simulink model "s_c_nbe_m32k"  (R2018a)
settings: Solver=VariableStepDiscrete  StartTime=0.0  StopTime=1000  RelTol=1e-3
undefined symbols (not defined in the file): fft_stages, n_taps, output_bits, pfb_coeff_gen_calc, xengbits
libraries: xbsIndex_r4 x23714, casper_library_misc x17, xps_library x4, casper_library_scopes x4, xbsReplacements_r4 x4
(part 153 of 171)

== system s_c_nbe_m32k/nb_pfb/pfb_fir_generic1/pfb_fir_taps/tap_delays/rep_web0 ==
  in : Inport
  bussify : Subsystem  mask(bus_create){inputNum=108}
      mask prompts: inputNum "Number of inputs:"
      mask init:
      | bus_create_init(gcb,...
      |     'inputNum', inputNum);
  din0_0 : xbsIndex_r4/Delay  rst=off  infoeditControl=Selection of Reset will increase slice count due to use of real FFs and instead of SRLs  en=off  latency=1  reg_retiming=off  dbl_ovrd=off  block_type=delay
  din0_1 : xbsIndex_r4/Delay  rst=off  infoeditControl=Selection of Reset will increase slice count due to use of real FFs and instead of SRLs  en=off  latency=1  reg_retiming=off  dbl_ovrd=off  block_type=delay
  din0_2 : xbsIndex_r4/Delay  rst=off  infoeditControl=Selection of Reset will increase slice count due to use of real FFs and instead of SRLs  en=off  latency=1  reg_retiming=off  dbl_ovrd=off  block_type=delay
  din1_{0..11} (12 alike) : xbsIndex_r4/Delay  rst=off  infoeditControl=Selection of Reset will increase slice count due to use of real FFs and instead of SRLs  en=off  latency=1  reg_retiming=off  dbl_ovrd=off  block_type=delay
  din2_{0..47} (48 alike) : xbsIndex_r4/Delay  rst=off  infoeditControl=Selection of Reset will increase slice count due to use of real FFs and instead of SRLs  en=off  latency=1  reg_retiming=off  dbl_ovrd=off  block_type=delay
  din3_{0..107} (108 alike) : xbsIndex_r4/Delay  rst=off  infoeditControl=Selection of Reset will increase slice count due to use of real FFs and instead of SRLs  en=off  latency=1  reg_retiming=off  dbl_ovrd=off  block_type=delay
  out : Outport
  wires:
  in/1 -> din0_0/1, din0_1/1, din0_2/1
  din0_0/1 -> din1_0/1, din1_3/1, din1_6/1, din1_9/1
  din0_1/1 -> din1_1/1, din1_4/1, din1_7/1, din1_10/1
  din0_2/1 -> din1_2/1, din1_5/1, din1_8/1, din1_11/1
  din1_0/1 -> din2_0/1, din2_12/1, din2_24/1, din2_36/1
  din1_1/1 -> din2_1/1, din2_13/1, din2_25/1, din2_37/1
  din1_2/1 -> din2_2/1, din2_14/1, din2_26/1, din2_38/1
  din1_3/1 -> din2_3/1, din2_15/1, din2_27/1, din2_39/1
  din1_4/1 -> din2_4/1, din2_16/1, din2_28/1, din2_40/1
  din1_5/1 -> din2_5/1, din2_17/1, din2_29/1, din2_41/1
  din1_6/1 -> din2_6/1, din2_18/1, din2_30/1, din2_42/1
  din1_7/1 -> din2_7/1, din2_19/1, din2_31/1, din2_43/1
  din1_8/1 -> din2_8/1, din2_20/1, din2_32/1, din2_44/1
  din1_9/1 -> din2_9/1, din2_21/1, din2_33/1, din2_45/1
  din1_10/1 -> din2_10/1, din2_22/1, din2_34/1, din2_46/1
  din1_11/1 -> din2_11/1, din2_23/1, din2_35/1, din2_47/1
  din2_0/1 -> din3_0/1, din3_48/1, din3_96/1
  din2_1/1 -> din3_1/1, din3_49/1, din3_97/1
  din2_2/1 -> din3_2/1, din3_50/1, din3_98/1
  din2_3/1 -> din3_3/1, din3_51/1, din3_99/1
  din2_4/1 -> din3_4/1, din3_52/1, din3_100/1
  din2_5/1 -> din3_5/1, din3_53/1, din3_101/1
  din2_6/1 -> din3_6/1, din3_54/1, din3_102/1
  din2_7/1 -> din3_7/1, din3_55/1, din3_103/1
  din2_8/1 -> din3_8/1, din3_56/1, din3_104/1
  din2_9/1 -> din3_9/1, din3_57/1, din3_105/1
  din2_10/1 -> din3_10/1, din3_58/1, din3_106/1
  din2_11/1 -> din3_11/1, din3_59/1, din3_107/1
  din2_12/1 -> din3_12/1, din3_60/1
  din2_13/1 -> din3_13/1, din3_61/1
  din2_14/1 -> din3_14/1, din3_62/1
  din2_15/1 -> din3_15/1, din3_63/1
  din2_16/1 -> din3_16/1, din3_64/1
  din2_17/1 -> din3_17/1, din3_65/1
  din2_18/1 -> din3_18/1, din3_66/1
  din2_19/1 -> din3_19/1, din3_67/1
  din2_20/1 -> din3_20/1, din3_68/1
  din2_21/1 -> din3_21/1, din3_69/1
  din2_22/1 -> din3_22/1, din3_70/1
  din2_23/1 -> din3_23/1, din3_71/1
  din2_24/1 -> din3_24/1, din3_72/1
  din2_25/1 -> din3_25/1, din3_73/1
  din2_26/1 -> din3_26/1, din3_74/1
  din2_27/1 -> din3_27/1, din3_75/1
  din2_28/1 -> din3_28/1, din3_76/1
  din2_29/1 -> din3_29/1, din3_77/1
  din2_30/1 -> din3_30/1, din3_78/1
  din2_31/1 -> din3_31/1, din3_79/1
  din2_32/1 -> din3_32/1, din3_80/1
  din2_33/1 -> din3_33/1, din3_81/1
  din2_34/1 -> din3_34/1, din3_82/1
  din2_35/1 -> din3_35/1, din3_83/1
  din2_36/1 -> din3_36/1, din3_84/1
  din2_37/1 -> din3_37/1, din3_85/1
  din2_38/1 -> din3_38/1, din3_86/1
  din2_39/1 -> din3_39/1, din3_87/1
  din2_40/1 -> din3_40/1, din3_88/1
  din2_41/1 -> din3_41/1, din3_89/1
  din2_42/1 -> din3_42/1, din3_90/1
  din2_43/1 -> din3_43/1, din3_91/1
  din2_44/1 -> din3_44/1, din3_92/1
  din2_45/1 -> din3_45/1, din3_93/1
  din2_46/1 -> din3_46/1, din3_94/1
  din2_47/1 -> din3_47/1, din3_95/1
  din3_0/1 -> bussify/1(in1)
  din3_1/1 -> bussify/2(in2)
  din3_2/1 -> bussify/3(in3)
  din3_3/1 -> bussify/4(in4)
  din3_4/1 -> bussify/5(in5)
  din3_5/1 -> bussify/6(in6)
  din3_6/1 -> bussify/7(in7)
  din3_7/1 -> bussify/8(in8)
  din3_8/1 -> bussify/9(in9)
  din3_9/1 -> bussify/10(in10)
  din3_10/1 -> bussify/11(in11)
  din3_11/1 -> bussify/12(in12)
  din3_12/1 -> bussify/13(in13)
  din3_13/1 -> bussify/14(in14)
  din3_14/1 -> bussify/15(in15)
  din3_15/1 -> bussify/16(in16)
  din3_16/1 -> bussify/17(in17)
  din3_17/1 -> bussify/18(in18)
  din3_18/1 -> bussify/19(in19)
  din3_19/1 -> bussify/20(in20)
  din3_20/1 -> bussify/21(in21)
  din3_21/1 -> bussify/22(in22)
  din3_22/1 -> bussify/23(in23)
  din3_23/1 -> bussify/24(in24)
  din3_24/1 -> bussify/25(in25)
  din3_25/1 -> bussify/26(in26)
  din3_26/1 -> bussify/27(in27)
  din3_27/1 -> bussify/28(in28)
  din3_28/1 -> bussify/29(in29)
  din3_29/1 -> bussify/30(in30)
  din3_30/1 -> bussify/31(in31)
  din3_31/1 -> bussify/32(in32)
  din3_32/1 -> bussify/33(in33)
  din3_33/1 -> bussify/34(in34)
  din3_34/1 -> bussify/35(in35)
  din3_35/1 -> bussify/36(in36)
  din3_36/1 -> bussify/37(in37)
  din3_37/1 -> bussify/38(in38)
  din3_38/1 -> bussify/39(in39)
  din3_39/1 -> bussify/40(in40)
  din3_40/1 -> bussify/41(in41)
  din3_41/1 -> bussify/42(in42)
  din3_42/1 -> bussify/43(in43)
  din3_43/1 -> bussify/44(in44)
  din3_44/1 -> bussify/45(in45)
  din3_45/1 -> bussify/46(in46)
  din3_46/1 -> bussify/47(in47)
  din3_47/1 -> bussify/48(in48)
  din3_48/1 -> bussify/49(in49)
  din3_49/1 -> bussify/50(in50)
  din3_50/1 -> bussify/51(in51)
  din3_51/1 -> bussify/52(in52)
  din3_52/1 -> bussify/53(in53)
  din3_53/1 -> bussify/54(in54)
  din3_54/1 -> bussify/55(in55)
  din3_55/1 -> bussify/56(in56)
  din3_56/1 -> bussify/57(in57)
  din3_57/1 -> bussify/58(in58)
  din3_58/1 -> bussify/59(in59)
  din3_59/1 -> bussify/60(in60)
  din3_60/1 -> bussify/61(in61)
  din3_61/1 -> bussify/62(in62)
  din3_62/1 -> bussify/63(in63)
  din3_63/1 -> bussify/64(in64)
  din3_64/1 -> bussify/65(in65)
  din3_65/1 -> bussify/66(in66)
  din3_66/1 -> bussify/67(in67)
  din3_67/1 -> bussify/68(in68)
  din3_68/1 -> bussify/69(in69)
  din3_69/1 -> bussify/70(in70)
  din3_70/1 -> bussify/71(in71)
  din3_71/1 -> bussify/72(in72)
  din3_72/1 -> bussify/73(in73)
  din3_73/1 -> bussify/74(in74)
  din3_74/1 -> bussify/75(in75)
  din3_75/1 -> bussify/76(in76)
  din3_76/1 -> bussify/77(in77)
  din3_77/1 -> bussify/78(in78)
  din3_78/1 -> bussify/79(in79)
  din3_79/1 -> bussify/80(in80)
  din3_80/1 -> bussify/81(in81)
  din3_81/1 -> bussify/82(in82)
  din3_82/1 -> bussify/83(in83)
  din3_83/1 -> bussify/84(in84)
  din3_84/1 -> bussify/85(in85)
  din3_85/1 -> bussify/86(in86)
  din3_86/1 -> bussify/87(in87)
  din3_87/1 -> bussify/88(in88)
  din3_88/1 -> bussify/89(in89)
  din3_89/1 -> bussify/90(in90)
  din3_90/1 -> bussify/91(in91)
  din3_91/1 -> bussify/92(in92)
  din3_92/1 -> bussify/93(in93)
  din3_93/1 -> bussify/94(in94)
  din3_94/1 -> bussify/95(in95)
  din3_95/1 -> bussify/96(in96)
  din3_96/1 -> bussify/97(in97)
  din3_97/1 -> bussify/98(in98)
  din3_98/1 -> bussify/99(in99)
  din3_99/1 -> bussify/100(in100)
  din3_100/1 -> bussify/101(in101)
  din3_101/1 -> bussify/102(in102)
  din3_102/1 -> bussify/103(in103)
  din3_103/1 -> bussify/104(in104)
  din3_104/1 -> bussify/105(in105)
  din3_105/1 -> bussify/106(in106)
  din3_106/1 -> bussify/107(in107)
  din3_107/1 -> bussify/108(in108)
  bussify/1(bus_out) -> out/1

== system s_c_nbe_m32k/nb_pfb/pfb_fir_generic2/pfb_fir_coeff_gen/munge/join ==
  in1 : Inport
  in2 : Inport  Port=2
  concatenate : xbsIndex_r4/Concat  num_inputs=2  dbl_ovrd=off  block_type=concat
  reinterpret1 : xbsIndex_r4/Reinterpret  force_arith_type=on  arith_type=Unsigned  force_bin_pt=on  bin_pt=0  block_type=reinterpret
      settings: infoedit="Changes signal type without altering the binary representation.   You can changed the signal between signed and unsigned, and relocate the binary point.<br><br>Hardware notes: In hardware this block costs nothing.<br><br>Example:  Suppose the input is 6 bits wide, signed, with 2 fractional bits, and the output is forced to unsigned with 0 fractional bits.  Then an input of -2.0 (1110.00 in binary 2's complement) becomes an output of 56 (111000 in binary)."
  reinterpret2 : xbsIndex_r4/Reinterpret  force_arith_type=on  arith_type=Unsigned  force_bin_pt=on  bin_pt=0  block_type=reinterpret
      settings: infoedit="Changes signal type without altering the binary representation.   You can changed the signal between signed and unsigned, and relocate the binary point.<br><br>Hardware notes: In hardware this block costs nothing.<br><br>Example:  Suppose the input is 6 bits wide, signed, with 2 fractional bits, and the output is forced to unsigned with 0 fractional bits.  Then an input of -2.0 (1110.00 in binary 2's complement) becomes an output of 56 (111000 in binary)."
  bus_out : Outport
  wires:
  concatenate/1 -> bus_out/1
  in1/1 -> reinterpret1/1
  reinterpret1/1 -> concatenate/1
  in2/1 -> reinterpret2/1
  reinterpret2/1 -> concatenate/2

== system s_c_nbe_m32k/nb_pfb/pfb_fir_generic2/pfb_fir_coeff_gen/munge/split ==
  bus_in : Inport
  reinterpret1 : xbsIndex_r4/Reinterpret  force_arith_type=on  arith_type=Unsigned  force_bin_pt=on  bin_pt=0  block_type=reinterpret
  reinterpret2 : xbsIndex_r4/Reinterpret  force_arith_type=on  arith_type=Unsigned  force_bin_pt=on  bin_pt=0  block_type=reinterpret
  slice1 : xbsIndex_r4/Slice  nbits=18  boolean_output=off  mode=Upper Bit Location + Width  bit1=-18  base1=MSB of Input  bit0=0  base0=LSB of Input  dbl_ovrd=off  block_type=slice
  slice2 : xbsIndex_r4/Slice  nbits=18  boolean_output=off  mode=Upper Bit Location + Width  bit1=0  base1=MSB of Input  bit0=0  base0=LSB of Input  dbl_ovrd=off  block_type=slice
  msb_out2 : Outport
  lsb_out1 : Outport  Port=2
  wires:
  bus_in/1 -> slice2/1, slice1/1
  slice2/1 -> reinterpret2/1
  reinterpret2/1 -> msb_out2/1
  slice1/1 -> reinterpret1/1
  reinterpret1/1 -> lsb_out1/1

== system s_c_nbe_m32k/nb_pfb/pfb_fir_generic2/pfb_fir_coeff_gen/rom/A_bussify0 ==
  in1 : Inport
  in2 : Inport  Port=2
  in3 : Inport  Port=3
  in4 : Inport  Port=4
  in5 : Inport  Port=5
  in6 : Inport  Port=6
  in7 : Inport  Port=7
  in8 : Inport  Port=8
  in9 : Inport  Port=9
  in10 : Inport  Port=10
  in11 : Inport  Port=11
  in12 : Inport  Port=12
  in13 : Inport  Port=13
  in14 : Inport  Port=14
  in15 : Inport  Port=15
  in16 : Inport  Port=16
  in17 : Inport  Port=17
  in18 : Inport  Port=18
  in19 : Inport  Port=19
  in20 : Inport  Port=20
  in21 : Inport  Port=21
  in22 : Inport  Port=22
  in23 : Inport  Port=23
  in24 : Inport  Port=24
  in25 : Inport  Port=25
  in26 : Inport  Port=26
  in27 : Inport  Port=27
  in28 : Inport  Port=28
  in29 : Inport  Port=29
  in30 : Inport  Port=30
  in31 : Inport  Port=31
  in32 : Inport  Port=32
  in33 : Inport  Port=33
  in34 : Inport  Port=34
  in35 : Inport  Port=35
  in36 : Inport  Port=36
  concatenate : xbsIndex_r4/Concat  num_inputs=36  dbl_ovrd=off  block_type=concat
  reinterpret{1..36} (36 alike) : xbsIndex_r4/Reinterpret  force_arith_type=on  arith_type=Unsigned  force_bin_pt=on  bin_pt=0  block_type=reinterpret
      reinterpret1 settings: infoedit="Changes signal type without altering the binary representation.   You can changed the signal between signed and unsigned, and relocate the binary point.<br><br>Hardware notes: In hardware this block costs nothing.<br><br>Example:  Suppose the input is 6 bits wide, signed, with 2 fractional bits, and the output is forced to unsigned with 0 fractional bits.  Then an input of -2.0 (1110.00 in binary 2's complement) becomes an output of 56 (111000 in binary)."
      reinterpret2 settings: infoedit="Changes signal type without altering the binary representation.   You can changed the signal between signed and unsigned, and relocate the binary point.<br><br>Hardware notes: In hardware this block costs nothing.<br><br>Example:  Suppose the input is 6 bits wide, signed, with 2 fractional bits, and the output is forced to unsigned with 0 fractional bits.  Then an input of -2.0 (1110.00 in binary 2's complement) becomes an output of 56 (111000 in binary)."
  bus_out : Outport
  wires:
  concatenate/1 -> bus_out/1
  in1/1 -> reinterpret1/1
  reinterpret1/1 -> concatenate/1
  in2/1 -> reinterpret2/1
  reinterpret2/1 -> concatenate/2
  in3/1 -> reinterpret3/1
  reinterpret3/1 -> concatenate/3
  in4/1 -> reinterpret4/1
  reinterpret4/1 -> concatenate/4
  in5/1 -> reinterpret5/1
  reinterpret5/1 -> concatenate/5
  in6/1 -> reinterpret6/1
  reinterpret6/1 -> concatenate/6
  in7/1 -> reinterpret7/1
  reinterpret7/1 -> concatenate/7
  in8/1 -> reinterpret8/1
  reinterpret8/1 -> concatenate/8
  in9/1 -> reinterpret9/1
  reinterpret9/1 -> concatenate/9
  in10/1 -> reinterpret10/1
  reinterpret10/1 -> concatenate/10
  in11/1 -> reinterpret11/1
  reinterpret11/1 -> concatenate/11
  in12/1 -> reinterpret12/1
  reinterpret12/1 -> concatenate/12
  in13/1 -> reinterpret13/1
  reinterpret13/1 -> concatenate/13
  in14/1 -> reinterpret14/1
  reinterpret14/1 -> concatenate/14
  in15/1 -> reinterpret15/1
  reinterpret15/1 -> concatenate/15
  in16/1 -> reinterpret16/1
  reinterpret16/1 -> concatenate/16
  in17/1 -> reinterpret17/1
  reinterpret17/1 -> concatenate/17
  in18/1 -> reinterpret18/1
  reinterpret18/1 -> concatenate/18
  in19/1 -> reinterpret19/1
  reinterpret19/1 -> concatenate/19
  in20/1 -> reinterpret20/1
  reinterpret20/1 -> concatenate/20
  in21/1 -> reinterpret21/1
  reinterpret21/1 -> concatenate/21
  in22/1 -> reinterpret22/1
  reinterpret22/1 -> concatenate/22
  in23/1 -> reinterpret23/1
  reinterpret23/1 -> concatenate/23
  in24/1 -> reinterpret24/1
  reinterpret24/1 -> concatenate/24
  in25/1 -> reinterpret25/1
  reinterpret25/1 -> concatenate/25
  in26/1 -> reinterpret26/1
  reinterpret26/1 -> concatenate/26
  in27/1 -> reinterpret27/1
  reinterpret27/1 -> concatenate/27
  in28/1 -> reinterpret28/1
  reinterpret28/1 -> concatenate/28
  in29/1 -> reinterpret29/1
  reinterpret29/1 -> concatenate/29
  in30/1 -> reinterpret30/1
  reinterpret30/1 -> concatenate/30
  in31/1 -> reinterpret31/1
  reinterpret31/1 -> concatenate/31
  in32/1 -> reinterpret32/1
  reinterpret32/1 -> concatenate/32
  in33/1 -> reinterpret33/1
  reinterpret33/1 -> concatenate/33
  in34/1 -> reinterpret34/1
  reinterpret34/1 -> concatenate/34
  in35/1 -> reinterpret35/1
  reinterpret35/1 -> concatenate/35
  in36/1 -> reinterpret36/1
  reinterpret36/1 -> concatenate/36

== system s_c_nbe_m32k/nb_pfb/pfb_fir_generic2/pfb_fir_coeff_gen/rom/B_bussify0 ==
  in1 : Inport
  in2 : Inport  Port=2
  in3 : Inport  Port=3
  in4 : Inport  Port=4
  in5 : Inport  Port=5
  in6 : Inport  Port=6
  in7 : Inport  Port=7
  in8 : Inport  Port=8
  in9 : Inport  Port=9
  in10 : Inport  Port=10
  in11 : Inport  Port=11
  in12 : Inport  Port=12
  in13 : Inport  Port=13
  in14 : Inport  Port=14
  in15 : Inport  Port=15
  in16 : Inport  Port=16
  in17 : Inport  Port=17
  in18 : Inport  Port=18
  in19 : Inport  Port=19
  in20 : Inport  Port=20
  in21 : Inport  Port=21
  in22 : Inport  Port=22
  in23 : Inport  Port=23
  in24 : Inport  Port=24
  in25 : Inport  Port=25
  in26 : Inport  Port=26
  in27 : Inport  Port=27
  in28 : Inport  Port=28
  in29 : Inport  Port=29
  in30 : Inport  Port=30
  in31 : Inport  Port=31
  in32 : Inport  Port=32
  in33 : Inport  Port=33
  in34 : Inport  Port=34
  in35 : Inport  Port=35
  in36 : Inport  Port=36
  concatenate : xbsIndex_r4/Concat  num_inputs=36  dbl_ovrd=off  block_type=concat
  reinterpret{1..36} (36 alike) : xbsIndex_r4/Reinterpret  force_arith_type=on  arith_type=Unsigned  force_bin_pt=on  bin_pt=0  block_type=reinterpret
      reinterpret1 settings: infoedit="Changes signal type without altering the binary representation.   You can changed the signal between signed and unsigned, and relocate the binary point.<br><br>Hardware notes: In hardware this block costs nothing.<br><br>Example:  Suppose the input is 6 bits wide, signed, with 2 fractional bits, and the output is forced to unsigned with 0 fractional bits.  Then an input of -2.0 (1110.00 in binary 2's complement) becomes an output of 56 (111000 in binary)."
      reinterpret2 settings: infoedit="Changes signal type without altering the binary representation.   You can changed the signal between signed and unsigned, and relocate the binary point.<br><br>Hardware notes: In hardware this block costs nothing.<br><br>Example:  Suppose the input is 6 bits wide, signed, with 2 fractional bits, and the output is forced to unsigned with 0 fractional bits.  Then an input of -2.0 (1110.00 in binary 2's complement) becomes an output of 56 (111000 in binary)."
  bus_out : Outport
  wires:
  concatenate/1 -> bus_out/1
  in1/1 -> reinterpret1/1
  reinterpret1/1 -> concatenate/1
  in2/1 -> reinterpret2/1
  reinterpret2/1 -> concatenate/2
  in3/1 -> reinterpret3/1
  reinterpret3/1 -> concatenate/3
  in4/1 -> reinterpret4/1
  reinterpret4/1 -> concatenate/4
  in5/1 -> reinterpret5/1
  reinterpret5/1 -> concatenate/5
  in6/1 -> reinterpret6/1
  reinterpret6/1 -> concatenate/6
  in7/1 -> reinterpret7/1
  reinterpret7/1 -> concatenate/7
  in8/1 -> reinterpret8/1
  reinterpret8/1 -> concatenate/8
  in9/1 -> reinterpret9/1
  reinterpret9/1 -> concatenate/9
  in10/1 -> reinterpret10/1
  reinterpret10/1 -> concatenate/10
  in11/1 -> reinterpret11/1
  reinterpret11/1 -> concatenate/11
  in12/1 -> reinterpret12/1
  reinterpret12/1 -> concatenate/12
  in13/1 -> reinterpret13/1
  reinterpret13/1 -> concatenate/13
  in14/1 -> reinterpret14/1
  reinterpret14/1 -> concatenate/14
  in15/1 -> reinterpret15/1
  reinterpret15/1 -> concatenate/15
  in16/1 -> reinterpret16/1
  reinterpret16/1 -> concatenate/16
  in17/1 -> reinterpret17/1
  reinterpret17/1 -> concatenate/17
  in18/1 -> reinterpret18/1
  reinterpret18/1 -> concatenate/18
  in19/1 -> reinterpret19/1
  reinterpret19/1 -> concatenate/19
  in20/1 -> reinterpret20/1
  reinterpret20/1 -> concatenate/20
  in21/1 -> reinterpret21/1
  reinterpret21/1 -> concatenate/21
  in22/1 -> reinterpret22/1
  reinterpret22/1 -> concatenate/22
  in23/1 -> reinterpret23/1
  reinterpret23/1 -> concatenate/23
  in24/1 -> reinterpret24/1
  reinterpret24/1 -> concatenate/24
  in25/1 -> reinterpret25/1
  reinterpret25/1 -> concatenate/25
  in26/1 -> reinterpret26/1
  reinterpret26/1 -> concatenate/26
  in27/1 -> reinterpret27/1
  reinterpret27/1 -> concatenate/27
  in28/1 -> reinterpret28/1
  reinterpret28/1 -> concatenate/28
  in29/1 -> reinterpret29/1
  reinterpret29/1 -> concatenate/29
  in30/1 -> reinterpret30/1
  reinterpret30/1 -> concatenate/30
  in31/1 -> reinterpret31/1
  reinterpret31/1 -> concatenate/31
  in32/1 -> reinterpret32/1
  reinterpret32/1 -> concatenate/32
  in33/1 -> reinterpret33/1
  reinterpret33/1 -> concatenate/33
  in34/1 -> reinterpret34/1
  reinterpret34/1 -> concatenate/34
  in35/1 -> reinterpret35/1
  reinterpret35/1 -> concatenate/35
  in36/1 -> reinterpret36/1
  reinterpret36/1 -> concatenate/36

== system s_c_nbe_m32k/nb_pfb/pfb_fir_generic2/pfb_fir_coeff_gen/rom/debus_addra0 ==
  bus_in : Inport
  reinterpret{1..36} (36 alike) : xbsIndex_r4/Reinterpret  force_arith_type=on  arith_type=Unsigned  force_bin_pt=on  bin_pt=0  block_type=reinterpret
  slice1 : xbsIndex_r4/Slice  nbits=15  boolean_output=off  mode=Upper Bit Location + Width  bit1=-525  base1=MSB of Input  bit0=0  base0=LSB of Input  dbl_ovrd=off  block_type=slice
  slice10 : xbsIndex_r4/Slice  nbits=15  boolean_output=off  mode=Upper Bit Location + Width  bit1=-390  base1=MSB of Input  bit0=0  base0=LSB of Input  dbl_ovrd=off  block_type=slice
  slice11 : xbsIndex_r4/Slice  nbits=15  boolean_output=off  mode=Upper Bit Location + Width  bit1=-375  base1=MSB of Input  bit0=0  base0=LSB of Input  dbl_ovrd=off  block_type=slice
  slice12 : xbsIndex_r4/Slice  nbits=15  boolean_output=off  mode=Upper Bit Location + Width  bit1=-360  base1=MSB of Input  bit0=0  base0=LSB of Input  dbl_ovrd=off  block_type=slice
  slice13 : xbsIndex_r4/Slice  nbits=15  boolean_output=off  mode=Upper Bit Location + Width  bit1=-345  base1=MSB of Input  bit0=0  base0=LSB of Input  dbl_ovrd=off  block_type=slice
  slice14 : xbsIndex_r4/Slice  nbits=15  boolean_output=off  mode=Upper Bit Location + Width  bit1=-330  base1=MSB of Input  bit0=0  base0=LSB of Input  dbl_ovrd=off  block_type=slice
  slice15 : xbsIndex_r4/Slice  nbits=15  boolean_output=off  mode=Upper Bit Location + Width  bit1=-315  base1=MSB of Input  bit0=0  base0=LSB of Input  dbl_ovrd=off  block_type=slice
  slice16 : xbsIndex_r4/Slice  nbits=15  boolean_output=off  mode=Upper Bit Location + Width  bit1=-300  base1=MSB of Input  bit0=0  base0=LSB of Input  dbl_ovrd=off  block_type=slice
  slice17 : xbsIndex_r4/Slice  nbits=15  boolean_output=off  mode=Upper Bit Location + Width  bit1=-285  base1=MSB of Input  bit0=0  base0=LSB of Input  dbl_ovrd=off  block_type=slice
  slice18 : xbsIndex_r4/Slice  nbits=15  boolean_output=off  mode=Upper Bit Location + Width  bit1=-270  base1=MSB of Input  bit0=0  base0=LSB of Input  dbl_ovrd=off  block_type=slice
  slice19 : xbsIndex_r4/Slice  nbits=15  boolean_output=off  mode=Upper Bit Location + Width  bit1=-255  base1=MSB of Input  bit0=0  base0=LSB of Input  dbl_ovrd=off  block_type=slice
  slice2 : xbsIndex_r4/Slice  nbits=15  boolean_output=off  mode=Upper Bit Location + Width  bit1=-510  base1=MSB of Input  bit0=0  base0=LSB of Input  dbl_ovrd=off  block_type=slice
  slice20 : xbsIndex_r4/Slice  nbits=15  boolean_output=off  mode=Upper Bit Location + Width  bit1=-240  base1=MSB of Input  bit0=0  base0=LSB of Input  dbl_ovrd=off  block_type=slice
  slice21 : xbsIndex_r4/Slice  nbits=15  boolean_output=off  mode=Upper Bit Location + Width  bit1=-225  base1=MSB of Input  bit0=0  base0=LSB of Input  dbl_ovrd=off  block_type=slice
  slice22 : xbsIndex_r4/Slice  nbits=15  boolean_output=off  mode=Upper Bit Location + Width  bit1=-210  base1=MSB of Input  bit0=0  base0=LSB of Input  dbl_ovrd=off  block_type=slice
  slice23 : xbsIndex_r4/Slice  nbits=15  boolean_output=off  mode=Upper Bit Location + Width  bit1=-195  base1=MSB of Input  bit0=0  base0=LSB of Input  dbl_ovrd=off  block_type=slice
  slice24 : xbsIndex_r4/Slice  nbits=15  boolean_output=off  mode=Upper Bit Location + Width  bit1=-180  base1=MSB of Input  bit0=0  base0=LSB of Input  dbl_ovrd=off  block_type=slice
  slice25 : xbsIndex_r4/Slice  nbits=15  boolean_output=off  mode=Upper Bit Location + Width  bit1=-165  base1=MSB of Input  bit0=0  base0=LSB of Input  dbl_ovrd=off  block_type=slice
  slice26 : xbsIndex_r4/Slice  nbits=15  boolean_output=off  mode=Upper Bit Location + Width  bit1=-150  base1=MSB of Input  bit0=0  base0=LSB of Input  dbl_ovrd=off  block_type=slice
  slice27 : xbsIndex_r4/Slice  nbits=15  boolean_output=off  mode=Upper Bit Location + Width  bit1=-135  base1=MSB of Input  bit0=0  base0=LSB of Input  dbl_ovrd=off  block_type=slice
  slice28 : xbsIndex_r4/Slice  nbits=15  boolean_output=off  mode=Upper Bit Location + Width  bit1=-120  base1=MSB of Input  bit0=0  base0=LSB of Input  dbl_ovrd=off  block_type=slice
  slice29 : xbsIndex_r4/Slice  nbits=15  boolean_output=off  mode=Upper Bit Location + Width  bit1=-105  base1=MSB of Input  bit0=0  base0=LSB of Input  dbl_ovrd=off  block_type=slice
  slice3 : xbsIndex_r4/Slice  nbits=15  boolean_output=off  mode=Upper Bit Location + Width  bit1=-495  base1=MSB of Input  bit0=0  base0=LSB of Input  dbl_ovrd=off  block_type=slice
  slice30 : xbsIndex_r4/Slice  nbits=15  boolean_output=off  mode=Upper Bit Location + Width  bit1=-90  base1=MSB of Input  bit0=0  base0=LSB of Input  dbl_ovrd=off  block_type=slice
  slice31 : xbsIndex_r4/Slice  nbits=15  boolean_output=off  mode=Upper Bit Location + Width  bit1=-75  base1=MSB of Input  bit0=0  base0=LSB of Input  dbl_ovrd=off  block_type=slice
  slice32 : xbsIndex_r4/Slice  nbits=15  boolean_output=off  mode=Upper Bit Location + Width  bit1=-60  base1=MSB of Input  bit0=0  base0=LSB of Input  dbl_ovrd=off  block_type=slice
  slice33 : xbsIndex_r4/Slice  nbits=15  boolean_output=off  mode=Upper Bit Location + Width  bit1=-45  base1=MSB of Input  bit0=0  base0=LSB of Input  dbl_ovrd=off  block_type=slice
  slice34 : xbsIndex_r4/Slice  nbits=15  boolean_output=off  mode=Upper Bit Location + Width  bit1=-30  base1=MSB of Input  bit0=0  base0=LSB of Input  dbl_ovrd=off  block_type=slice
  slice35 : xbsIndex_r4/Slice  nbits=15  boolean_output=off  mode=Upper Bit Location + Width  bit1=-15  base1=MSB of Input  bit0=0  base0=LSB of Input  dbl_ovrd=off  block_type=slice
  slice36 : xbsIndex_r4/Slice  nbits=15  boolean_output=off  mode=Upper Bit Location + Width  bit1=0  base1=MSB of Input  bit0=0  base0=LSB of Input  dbl_ovrd=off  block_type=slice
  slice4 : xbsIndex_r4/Slice  nbits=15  boolean_output=off  mode=Upper Bit Location + Width  bit1=-480  base1=MSB of Input  bit0=0  base0=LSB of Input  dbl_ovrd=off  block_type=slice
  slice5 : xbsIndex_r4/Slice  nbits=15  boolean_output=off  mode=Upper Bit Location + Width  bit1=-465  base1=MSB of Input  bit0=0  base0=LSB of Input  dbl_ovrd=off  block_type=slice
  slice6 : xbsIndex_r4/Slice  nbits=15  boolean_output=off  mode=Upper Bit Location + Width  bit1=-450  base1=MSB of Input  bit0=0  base0=LSB of Input  dbl_ovrd=off  block_type=slice
  slice7 : xbsIndex_r4/Slice  nbits=15  boolean_output=off  mode=Upper Bit Location + Width  bit1=-435  base1=MSB of Input  bit0=0  base0=LSB of Input  dbl_ovrd=off  block_type=slice
  slice8 : xbsIndex_r4/Slice  nbits=15  boolean_output=off  mode=Upper Bit Location + Width  bit1=-420  base1=MSB of Input  bit0=0  base0=LSB of Input  dbl_ovrd=off  block_type=slice
  slice9 : xbsIndex_r4/Slice  nbits=15  boolean_output=off  mode=Upper Bit Location + Width  bit1=-405  base1=MSB of Input  bit0=0  base0=LSB of Input  dbl_ovrd=off  block_type=slice
  msb_out36 : Outport
  out35 : Outport  Port=2
  out34 : Outport  Port=3
  out33 : Outport  Port=4
  out32 : Outport  Port=5
  out31 : Outport  Port=6
  out30 : Outport  Port=7
  out29 : Outport  Port=8
  out28 : Outport  Port=9
  out27 : Outport  Port=10
  out26 : Outport  Port=11
  out25 : Outport  Port=12
  out24 : Outport  Port=13
  out23 : Outport  Port=14
  out22 : Outport  Port=15
  out21 : Outport  Port=16
  out20 : Outport  Port=17
  out19 : Outport  Port=18
  out18 : Outport  Port=19
  out17 : Outport  Port=20
  out16 : Outport  Port=21
  out15 : Outport  Port=22
  out14 : Outport  Port=23
  out13 : Outport  Port=24
  out12 : Outport  Port=25
  out11 : Outport  Port=26
  out10 : Outport  Port=27
  out9 : Outport  Port=28
  out8 : Outport  Port=29
  out7 : Outport  Port=30
  out6 : Outport  Port=31
  out5 : Outport  Port=32
  out4 : Outport  Port=33
  out3 : Outport  Port=34
  out2 : Outport  Port=35
  lsb_out1 : Outport  Port=36
  wires:
  bus_in/1 -> slice36/1, slice35/1, slice34/1, slice33/1, slice32/1, slice31/1, slice30/1, slice29/1, slice28/1, slice27/1, slice26/1, slice25/1, slice24/1, slice23/1, slice22/1, slice21/1, slice20/1, slice19/1, slice18/1, slice17/1, slice16/1, slice15/1, slice14/1, slice13/1, slice12/1, slice11/1, slice10/1, slice9/1, slice8/1, slice7/1, slice6/1, slice5/1, slice4/1, slice3/1, slice2/1, slice1/1
  slice36/1 -> reinterpret36/1
  reinterpret36/1 -> msb_out36/1
  slice35/1 -> reinterpret35/1
  reinterpret35/1 -> out35/1
  slice34/1 -> reinterpret34/1
  reinterpret34/1 -> out34/1
  slice33/1 -> reinterpret33/1
  reinterpret33/1 -> out33/1
  slice32/1 -> reinterpret32/1
  reinterpret32/1 -> out32/1
  slice31/1 -> reinterpret31/1
  reinterpret31/1 -> out31/1
  slice30/1 -> reinterpret30/1
  reinterpret30/1 -> out30/1
  slice29/1 -> reinterpret29/1
  reinterpret29/1 -> out29/1
  slice28/1 -> reinterpret28/1
  reinterpret28/1 -> out28/1
  slice27/1 -> reinterpret27/1
  reinterpret27/1 -> out27/1
  slice26/1 -> reinterpret26/1
  reinterpret26/1 -> out26/1
  slice25/1 -> reinterpret25/1
  reinterpret25/1 -> out25/1
  slice24/1 -> reinterpret24/1
  reinterpret24/1 -> out24/1
  slice23/1 -> reinterpret23/1
  reinterpret23/1 -> out23/1
  slice22/1 -> reinterpret22/1
  reinterpret22/1 -> out22/1
  slice21/1 -> reinterpret21/1
  reinterpret21/1 -> out21/1
  slice20/1 -> reinterpret20/1
  reinterpret20/1 -> out20/1
  slice19/1 -> reinterpret19/1
  reinterpret19/1 -> out19/1
  slice18/1 -> reinterpret18/1
  reinterpret18/1 -> out18/1
  slice17/1 -> reinterpret17/1
  reinterpret17/1 -> out17/1
  slice16/1 -> reinterpret16/1
  reinterpret16/1 -> out16/1
  slice15/1 -> reinterpret15/1
  reinterpret15/1 -> out15/1
  slice14/1 -> reinterpret14/1
  reinterpret14/1 -> out14/1
  slice13/1 -> reinterpret13/1
  reinterpret13/1 -> out13/1
  slice12/1 -> reinterpret12/1
  reinterpret12/1 -> out12/1
  slice11/1 -> reinterpret11/1
  reinterpret11/1 -> out11/1
  slice10/1 -> reinterpret10/1
  reinterpret10/1 -> out10/1
  slice9/1 -> reinterpret9/1
  reinterpret9/1 -> out9/1
  slice8/1 -> reinterpret8/1
  reinterpret8/1 -> out8/1
  slice7/1 -> reinterpret7/1
  reinterpret7/1 -> out7/1
  slice6/1 -> reinterpret6/1
  reinterpret6/1 -> out6/1
  slice5/1 -> reinterpret5/1
  reinterpret5/1 -> out5/1
  slice4/1 -> reinterpret4/1
  reinterpret4/1 -> out4/1
  slice3/1 -> reinterpret3/1
  reinterpret3/1 -> out3/1
  slice2/1 -> reinterpret2/1
  reinterpret2/1 -> out2/1
  slice1/1 -> reinterpret1/1
  reinterpret1/1 -> lsb_out1/1

== system s_c_nbe_m32k/nb_pfb/pfb_fir_generic2/pfb_fir_coeff_gen/rom/debus_addrb0 ==
  bus_in : Inport
  reinterpret{1..36} (36 alike) : xbsIndex_r4/Reinterpret  force_arith_type=on  arith_type=Unsigned  force_bin_pt=on  bin_pt=0  block_type=reinterpret
  slice1 : xbsIndex_r4/Slice  nbits=15  boolean_output=off  mode=Upper Bit Location + Width  bit1=-525  base1=MSB of Input  bit0=0  base0=LSB of Input  dbl_ovrd=off  block_type=slice
  slice10 : xbsIndex_r4/Slice  nbits=15  boolean_output=off  mode=Upper Bit Location + Width  bit1=-390  base1=MSB of Input  bit0=0  base0=LSB of Input  dbl_ovrd=off  block_type=slice
  slice11 : xbsIndex_r4/Slice  nbits=15  boolean_output=off  mode=Upper Bit Location + Width  bit1=-375  base1=MSB of Input  bit0=0  base0=LSB of Input  dbl_ovrd=off  block_type=slice
  slice12 : xbsIndex_r4/Slice  nbits=15  boolean_output=off  mode=Upper Bit Location + Width  bit1=-360  base1=MSB of Input  bit0=0  base0=LSB of Input  dbl_ovrd=off  block_type=slice
  slice13 : xbsIndex_r4/Slice  nbits=15  boolean_output=off  mode=Upper Bit Location + Width  bit1=-345  base1=MSB of Input  bit0=0  base0=LSB of Input  dbl_ovrd=off  block_type=slice
  slice14 : xbsIndex_r4/Slice  nbits=15  boolean_output=off  mode=Upper Bit Location + Width  bit1=-330  base1=MSB of Input  bit0=0  base0=LSB of Input  dbl_ovrd=off  block_type=slice
  slice15 : xbsIndex_r4/Slice  nbits=15  boolean_output=off  mode=Upper Bit Location + Width  bit1=-315  base1=MSB of Input  bit0=0  base0=LSB of Input  dbl_ovrd=off  block_type=slice
  slice16 : xbsIndex_r4/Slice  nbits=15  boolean_output=off  mode=Upper Bit Location + Width  bit1=-300  base1=MSB of Input  bit0=0  base0=LSB of Input  dbl_ovrd=off  block_type=slice
  slice17 : xbsIndex_r4/Slice  nbits=15  boolean_output=off  mode=Upper Bit Location + Width  bit1=-285  base1=MSB of Input  bit0=0  base0=LSB of Input  dbl_ovrd=off  block_type=slice
  slice18 : xbsIndex_r4/Slice  nbits=15  boolean_output=off  mode=Upper Bit Location + Width  bit1=-270  base1=MSB of Input  bit0=0  base0=LSB of Input  dbl_ovrd=off  block_type=slice
  slice19 : xbsIndex_r4/Slice  nbits=15  boolean_output=off  mode=Upper Bit Location + Width  bit1=-255  base1=MSB of Input  bit0=0  base0=LSB of Input  dbl_ovrd=off  block_type=slice
  slice2 : xbsIndex_r4/Slice  nbits=15  boolean_output=off  mode=Upper Bit Location + Width  bit1=-510  base1=MSB of Input  bit0=0  base0=LSB of Input  dbl_ovrd=off  block_type=slice
  slice20 : xbsIndex_r4/Slice  nbits=15  boolean_output=off  mode=Upper Bit Location + Width  bit1=-240  base1=MSB of Input  bit0=0  base0=LSB of Input  dbl_ovrd=off  block_type=slice
  slice21 : xbsIndex_r4/Slice  nbits=15  boolean_output=off  mode=Upper Bit Location + Width  bit1=-225  base1=MSB of Input  bit0=0  base0=LSB of Input  dbl_ovrd=off  block_type=slice
  slice22 : xbsIndex_r4/Slice  nbits=15  boolean_output=off  mode=Upper Bit Location + Width  bit1=-210  base1=MSB of Input  bit0=0  base0=LSB of Input  dbl_ovrd=off  block_type=slice
  slice23 : xbsIndex_r4/Slice  nbits=15  boolean_output=off  mode=Upper Bit Location + Width  bit1=-195  base1=MSB of Input  bit0=0  base0=LSB of Input  dbl_ovrd=off  block_type=slice
  slice24 : xbsIndex_r4/Slice  nbits=15  boolean_output=off  mode=Upper Bit Location + Width  bit1=-180  base1=MSB of Input  bit0=0  base0=LSB of Input  dbl_ovrd=off  block_type=slice
  slice25 : xbsIndex_r4/Slice  nbits=15  boolean_output=off  mode=Upper Bit Location + Width  bit1=-165  base1=MSB of Input  bit0=0  base0=LSB of Input  dbl_ovrd=off  block_type=slice
  slice26 : xbsIndex_r4/Slice  nbits=15  boolean_output=off  mode=Upper Bit Location + Width  bit1=-150  base1=MSB of Input  bit0=0  base0=LSB of Input  dbl_ovrd=off  block_type=slice
  slice27 : xbsIndex_r4/Slice  nbits=15  boolean_output=off  mode=Upper Bit Location + Width  bit1=-135  base1=MSB of Input  bit0=0  base0=LSB of Input  dbl_ovrd=off  block_type=slice
  slice28 : xbsIndex_r4/Slice  nbits=15  boolean_output=off  mode=Upper Bit Location + Width  bit1=-120  base1=MSB of Input  bit0=0  base0=LSB of Input  dbl_ovrd=off  block_type=slice
  slice29 : xbsIndex_r4/Slice  nbits=15  boolean_output=off  mode=Upper Bit Location + Width  bit1=-105  base1=MSB of Input  bit0=0  base0=LSB of Input  dbl_ovrd=off  block_type=slice
  slice3 : xbsIndex_r4/Slice  nbits=15  boolean_output=off  mode=Upper Bit Location + Width  bit1=-495  base1=MSB of Input  bit0=0  base0=LSB of Input  dbl_ovrd=off  block_type=slice
  slice30 : xbsIndex_r4/Slice  nbits=15  boolean_output=off  mode=Upper Bit Location + Width  bit1=-90  base1=MSB of Input  bit0=0  base0=LSB of Input  dbl_ovrd=off  block_type=slice
  slice31 : xbsIndex_r4/Slice  nbits=15  boolean_output=off  mode=Upper Bit Location + Width  bit1=-75  base1=MSB of Input  bit0=0  base0=LSB of Input  dbl_ovrd=off  block_type=slice
  slice32 : xbsIndex_r4/Slice  nbits=15  boolean_output=off  mode=Upper Bit Location + Width  bit1=-60  base1=MSB of Input  bit0=0  base0=LSB of Input  dbl_ovrd=off  block_type=slice
  slice33 : xbsIndex_r4/Slice  nbits=15  boolean_output=off  mode=Upper Bit Location + Width  bit1=-45  base1=MSB of Input  bit0=0  base0=LSB of Input  dbl_ovrd=off  block_type=slice
  slice34 : xbsIndex_r4/Slice  nbits=15  boolean_output=off  mode=Upper Bit Location + Width  bit1=-30  base1=MSB of Input  bit0=0  base0=LSB of Input  dbl_ovrd=off  block_type=slice
  slice35 : xbsIndex_r4/Slice  nbits=15  boolean_output=off  mode=Upper Bit Location + Width  bit1=-15  base1=MSB of Input  bit0=0  base0=LSB of Input  dbl_ovrd=off  block_type=slice
  slice36 : xbsIndex_r4/Slice  nbits=15  boolean_output=off  mode=Upper Bit Location + Width  bit1=0  base1=MSB of Input  bit0=0  base0=LSB of Input  dbl_ovrd=off  block_type=slice
  slice4 : xbsIndex_r4/Slice  nbits=15  boolean_output=off  mode=Upper Bit Location + Width  bit1=-480  base1=MSB of Input  bit0=0  base0=LSB of Input  dbl_ovrd=off  block_type=slice
  slice5 : xbsIndex_r4/Slice  nbits=15  boolean_output=off  mode=Upper Bit Location + Width  bit1=-465  base1=MSB of Input  bit0=0  base0=LSB of Input  dbl_ovrd=off  block_type=slice
  slice6 : xbsIndex_r4/Slice  nbits=15  boolean_output=off  mode=Upper Bit Location + Width  bit1=-450  base1=MSB of Input  bit0=0  base0=LSB of Input  dbl_ovrd=off  block_type=slice
  slice7 : xbsIndex_r4/Slice  nbits=15  boolean_output=off  mode=Upper Bit Location + Width  bit1=-435  base1=MSB of Input  bit0=0  base0=LSB of Input  dbl_ovrd=off  block_type=slice
  slice8 : xbsIndex_r4/Slice  nbits=15  boolean_output=off  mode=Upper Bit Location + Width  bit1=-420  base1=MSB of Input  bit0=0  base0=LSB of Input  dbl_ovrd=off  block_type=slice
  slice9 : xbsIndex_r4/Slice  nbits=15  boolean_output=off  mode=Upper Bit Location + Width  bit1=-405  base1=MSB of Input  bit0=0  base0=LSB of Input  dbl_ovrd=off  block_type=slice
  msb_out36 : Outport
  out35 : Outport  Port=2
  out34 : Outport  Port=3
  out33 : Outport  Port=4
  out32 : Outport  Port=5
  out31 : Outport  Port=6
  out30 : Outport  Port=7
  out29 : Outport  Port=8
  out28 : Outport  Port=9
  out27 : Outport  Port=10
  out26 : Outport  Port=11
  out25 : Outport  Port=12
  out24 : Outport  Port=13
  out23 : Outport  Port=14
  out22 : Outport  Port=15
  out21 : Outport  Port=16
  out20 : Outport  Port=17
  out19 : Outport  Port=18
  out18 : Outport  Port=19
  out17 : Outport  Port=20
  out16 : Outport  Port=21
  out15 : Outport  Port=22
  out14 : Outport  Port=23
  out13 : Outport  Port=24
  out12 : Outport  Port=25
  out11 : Outport  Port=26
  out10 : Outport  Port=27
  out9 : Outport  Port=28
  out8 : Outport  Port=29
  out7 : Outport  Port=30
  out6 : Outport  Port=31
  out5 : Outport  Port=32
  out4 : Outport  Port=33
  out3 : Outport  Port=34
  out2 : Outport  Port=35
  lsb_out1 : Outport  Port=36
  wires:
  bus_in/1 -> slice36/1, slice35/1, slice34/1, slice33/1, slice32/1, slice31/1, slice30/1, slice29/1, slice28/1, slice27/1, slice26/1, slice25/1, slice24/1, slice23/1, slice22/1, slice21/1, slice20/1, slice19/1, slice18/1, slice17/1, slice16/1, slice15/1, slice14/1, slice13/1, slice12/1, slice11/1, slice10/1, slice9/1, slice8/1, slice7/1, slice6/1, slice5/1, slice4/1, slice3/1, slice2/1, slice1/1
  slice36/1 -> reinterpret36/1
  reinterpret36/1 -> msb_out36/1
  slice35/1 -> reinterpret35/1
  reinterpret35/1 -> out35/1
  slice34/1 -> reinterpret34/1
  reinterpret34/1 -> out34/1
  slice33/1 -> reinterpret33/1
  reinterpret33/1 -> out33/1
  slice32/1 -> reinterpret32/1
  reinterpret32/1 -> out32/1
  slice31/1 -> reinterpret31/1
  reinterpret31/1 -> out31/1
  slice30/1 -> reinterpret30/1
  reinterpret30/1 -> out30/1
  slice29/1 -> reinterpret29/1
  reinterpret29/1 -> out29/1
  slice28/1 -> reinterpret28/1
  reinterpret28/1 -> out28/1
  slice27/1 -> reinterpret27/1
  reinterpret27/1 -> out27/1
  slice26/1 -> reinterpret26/1
  reinterpret26/1 -> out26/1
  slice25/1 -> reinterpret25/1
  reinterpret25/1 -> out25/1
  slice24/1 -> reinterpret24/1
  reinterpret24/1 -> out24/1
  slice23/1 -> reinterpret23/1
  reinterpret23/1 -> out23/1
  slice22/1 -> reinterpret22/1
  reinterpret22/1 -> out22/1
  slice21/1 -> reinterpret21/1
  reinterpret21/1 -> out21/1
  slice20/1 -> reinterpret20/1
  reinterpret20/1 -> out20/1
  slice19/1 -> reinterpret19/1
  reinterpret19/1 -> out19/1
  slice18/1 -> reinterpret18/1
  reinterpret18/1 -> out18/1
  slice17/1 -> reinterpret17/1
  reinterpret17/1 -> out17/1
  slice16/1 -> reinterpret16/1
  reinterpret16/1 -> out16/1
  slice15/1 -> reinterpret15/1
  reinterpret15/1 -> out15/1
  slice14/1 -> reinterpret14/1
  reinterpret14/1 -> out14/1
  slice13/1 -> reinterpret13/1
  reinterpret13/1 -> out13/1
  slice12/1 -> reinterpret12/1
  reinterpret12/1 -> out12/1
  slice11/1 -> reinterpret11/1
  reinterpret11/1 -> out11/1
  slice10/1 -> reinterpret10/1
  reinterpret10/1 -> out10/1
  slice9/1 -> reinterpret9/1
  reinterpret9/1 -> out9/1
  slice8/1 -> reinterpret8/1
  reinterpret8/1 -> out8/1
  slice7/1 -> reinterpret7/1
  reinterpret7/1 -> out7/1
  slice6/1 -> reinterpret6/1
  reinterpret6/1 -> out6/1
  slice5/1 -> reinterpret5/1
  reinterpret5/1 -> out5/1
  slice4/1 -> reinterpret4/1
  reinterpret4/1 -> out4/1
  slice3/1 -> reinterpret3/1
  reinterpret3/1 -> out3/1
  slice2/1 -> reinterpret2/1
  reinterpret2/1 -> out2/1
  slice1/1 -> reinterpret1/1
  reinterpret1/1 -> lsb_out1/1
